simulink model "smart_sensor"  (Simulink 7.0)
settings: Solver=FixedStepDiscrete  StartTime=0.0  StopTime=10.0  FixedStep=0.001  RelTol=1e-3
libraries: dsPICdrivers x8, simulink x1
settings Model: Creator=Zion  LastModifiedBy=Lubin
settings OptimizationCC: OptimizeModelRefInitCode=on  LifeSpan=1
settings HardwareCC: ProdBitPerInt=16  ProdEndianess=LittleEndian  ProdWordSize=16  ProdHWDeviceType=16-bit Generic  TargetHWDeviceType=32-bit Generic
settings RTWCC: SystemTargetFile=dspic.tlc  TemplateMakefile=dspic_pic30_gcc.tmf  PostCodeGenCommand=dsPIC_Compile()  Description=Embedded Target for Microchip dsPIC (real-time)  ProcessScript=dspic_make_rtw_hook
settings CodeAppCC: IgnoreCustomStorageClasses=off
settings STFCustomTargetCC: GenFloatMathFcnCalls=ANSI_C  ModelReferenceCompliant=off  IncludeMdlTerminateFcn=off  CombineOutputUpdateFcns=on  SuppressErrorStatus=on  ERTCustomFileBanners=on  SupportContinuousTime=off  SupportNonInlinedSFcns=off  SystemTargetFile=dspic.tlc
settings ERTTargetCC: GenFloatMathFcnCalls=ANSI_C  ModelReferenceCompliant=off  CompOptLevelCompliant=off  IncludeMdlTerminateFcn=off  SuppressErrorStatus=on  ModelStepFunctionPrototypeControlCompliant=off  InlinedParameterPlacement=NonHierarchical  ERTSrcFileBannerTemplate=dsPIC_code_template.cgt  ERTHdrFileBannerTemplate=dsPIC_code_template.cgt  ERTDataSrcFileTemplate=dsPIC_code_template.cgt  ERTDataHdrFileTemplate=dsPIC_code_template.cgt  ERTCustomFileTemplate=dsPIC_main.tlc
settings CustomProperty: DataType=string  Value=C:\PROGRA~1\MATLAB\R2007b\bin\win32\gmake

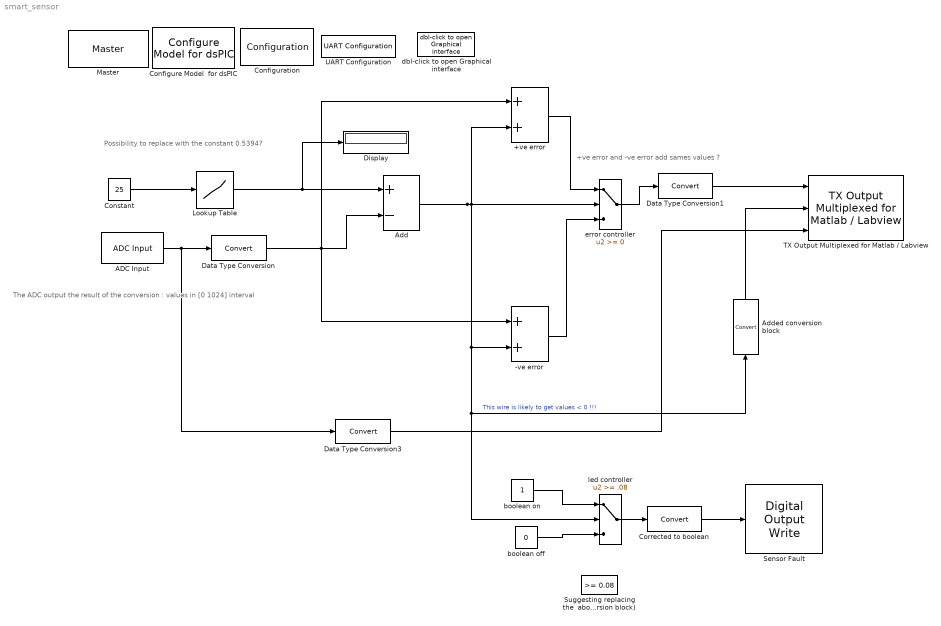
== system smart_sensor ==
  note: Possibility to replace with the constant 0.5394?
  note: The ADC output the
      | result of the conversion :
      | values in [0 1024] interval
  note: +ve error and -ve error add sames values ?
  +ve error : Sum  OutDataTypeMode=double  OutDataType=sfix(16)  OutScaling=2^-10
  -ve error : Sum  OutDataTypeMode=double  OutDataType=sfix(16)  OutScaling=2^-10
  ADC Input : dsPICdrivers/Peripheral I//O/ADC Input  Tag=dsPIC_ADC  Priority=5  ADC_TYPE=10 bits  ADC_MODE=Continuous sampling & get last channel value  NbrSampleStep=1  VoltRefpopup="AVdd  -  AVss"  OutFormatBitspopup=0000 00dd dddd dddd : Integer  InterruptPriority=6  ANCHANNELS=[0]  MaxName=ANmax = 1024  Rin=1e2  ADCS=1  SAMC=1  Temperature=25  SampleTime=-1  Status="OK  |  Tsmp=2.000e-007 |  T/Channel=2.600e-006 |  Tall=2.600e-006"
  Add : Sum  Inputs=+-  OutDataType=sfix(16)  OutScaling=2^-10
  Added conversion block : DataTypeConversion  Orientation=up  OutDataTypeMode=uint16  OutDataType=sfix(16)  OutScaling=2^0
  Configuration : dsPICdrivers/Configuration  SystemSampleTime=-1  double64=on
  Configure Model  for dsPIC : dsPICdrivers/Simulink Configuration/Configure Model  for dsPIC
  Constant : Constant  Value=25  OutDataTypeMode=double  OutDataType=sfix(16)  OutScaling=2^0
  Corrected to boolean : DataTypeConversion  OutDataTypeMode=boolean  OutDataType=sfix(16)  OutScaling=2^0
  Data Type Conversion : DataTypeConversion  OutDataTypeMode=double  OutDataType=sfix(16)  OutScaling=2^0
  Data Type Conversion1 : DataTypeConversion  OutDataTypeMode=uint16  OutDataType=sfix(16)  OutScaling=2^0
  Data Type Conversion3 : DataTypeConversion  OutDataTypeMode=uint16  OutDataType=sfix(16)  OutScaling=2^0
  Display : Display
  Lookup Table : Lookup  InputValues=[-55 23 150]  Table=[-1.1 .5 3]  LookUpMeth=Interpolation-Use End Values  OutDataTypeMode=double  OutDataType=sfix(16)  OutScaling=2^0
  Master : dsPICdrivers/Master  Tag=dsPIC_MASTER  Priority=1  TimeStepType=Timer1  picType=30f3011  fcy=5e6  Quartz_33f=5e6  PLLActive_33f=off  fcyDesired_33f=0  tmr1="[1  4999  0]"  tmr1Info="Time Step : 0.001  ;   Error : 0%  PR1=4999"  tmr2345="[0  0  0  0]"  tmr2345cfg=[-1 -1 -1 -1]  IOautoConf=on  typePort="[ 0   0   0   0   0   0   0   0   0   0   0   0   0   0   0   0   8   0   0   0   0   0   0   0   0   0   0   0   0   0   0   0   0   0   0   0   0   0   0   0   0   0   0   0   0   0   0   0   0   0   0   0   0   0   0   0   0   0   0   0   0   0   0   0  10   0   0   0   0   0   0   0   0   0   0   0   0   0   0   0   0   0   0   0   4   0   0   0   0   0   0   0   0   0   0   0   0   0   0   0   0   0   0   0   0   0   0   0   0   0   0   0 ]"  TRIS="[ 65535  65535  65535  65535  65534  65535  65535 ]"  ADPCFG=0  MasterBusyPort=None  MasterOverloadPort=None  FOSC=HS  TempProtection_33f=TEMP_ON  FPBOR=PBOR_OFF  PWRT=PWRT_OFF  MCLR=MCLR_DIS  PowerSave=off
  Sensor Fault : dsPICdrivers/Digital I//O/Digital Output Write  Tag=dsPIC_Digital_Output  Priority=5  PORT=E  Pin=[0 ]  Simultaneous=off  OrderingInOutPopup=None
  Suggesting replacing the  above blocks with this (replace also the conversion block) : simulink/Logic and Bit Operations/Compare To Constant  SystemSampleTime=-1  relop=>=  const=0.08  LogicOutDataTypeMode=boolean  ZeroCross=off
  TX Output Multiplexed for Matlab / Labview : dsPICdrivers/Serial PORT/TX Output Multiplexed for Matlab // Labview  Tag=dsPIC_TX_Multiplexed  Priority=5  UART=1  CleverSpreadingChk=on  CleverSpreading=1  CHANNEL=[0 1 2]  BUFFERSIZE=16  CHANNELBLOCKED=[]  CHANNELBLOCKED_BITEWISE=0  Status=OK
  UART Configuration : dsPICdrivers/Serial PORT/UART Configuration  Tag=dsPIC_config_UART  Priority=2  UART=2  proposed_BAUD=38400  ALT_TX_RX=on  TXInterruptPri=1  InterruptTxWhen=on TxBUF becoming empty  TXEN=off  RXInterruptPri=1  BAUD=38400  UxBRG=7  Info="UxBRG = 7   ||  Real Baud : 39063   ||  % error : 1.7253  ||  max 3.9063 Bytes / Step"  RealBaud=0
  boolean off : Constant  Value=0  OutDataTypeMode=double  OutDataType=sfix(16)  OutScaling=2^0
  boolean on : Constant  OutDataTypeMode=double  OutDataType=sfix(16)  OutScaling=2^0
  dbl-click to open Graphical interface : dsPICdrivers/Serial PORT/dbl-click to open Graphical interface  SystemSampleTime=-1
  error controller : Switch  OutDataTypeMode=double  OutDataType=sfix(16)  OutScaling=2^0
  led controller : Switch  Threshold=.08  OutDataTypeMode=double  OutDataType=sfix(16)  OutScaling=2^0
  wires:
  Constant/1 -> Lookup Table/1
  Lookup Table/1 -> Add/1, Display/1
  Add/1 -> +ve error/2, -ve error/2, led controller/2, Added conversion block/1, error controller/2  "This wire is likely to get values < 0 !!!"
  +ve error/1 -> error controller/1
  -ve error/1 -> error controller/3
  Data Type Conversion/1 -> Add/2, +ve error/1, -ve error/1
  ADC Input/1 -> Data Type Conversion/1, Data Type Conversion3/1
  error controller/1 -> Data Type Conversion1/1
  boolean on/1 -> led controller/1
  boolean off/1 -> led controller/3
  led controller/1 -> Corrected to boolean/1
  Corrected to boolean/1 -> Sensor Fault/1
  Data Type Conversion1/1 -> TX Output Multiplexed for Matlab / Labview/1
  Data Type Conversion3/1 -> TX Output Multiplexed for Matlab / Labview/3
  Added conversion block/1 -> TX Output Multiplexed for Matlab / Labview/2
